simulink model "Simulink_Validation_Two_Bus_OPF_DER_Constraints"  (R2023b)
settings: Solver=ode4  StartTime=0.0  StopTime=1  FixedStep=1e-6  RelTol=1e-3  EnableMultiTasking=on
libraries: spsRMSLib x7, rtlab x3, spsControlledCurrentSourceLib x3, spsThreePhaseParallelRLCLoadLib x3, spsLoadFlowBusLib x2, spsThreePhaseVIMeasurementLib x2, SignalEditorBlockLib x2, eeGeneralControl x1, spsGroundLib x1, spsThreePhasePISectionLineLib x1, spsThreePhaseSourceLib x1, spsThreePhaseDynamicLoadLib x1
Description:
  | Model of a simple control system for use iin training.
settings Model: Creator=Paul Baracos  LastModifiedBy=Ali
settings SolverCC: AlgebraicLoopSolver=TrustRegion  AutoInsertRateTranBlk=on
settings DataIOCC: LimitDataPoints=on  SaveFormat=Array  SignalLoggingSaveFormat=ModelDataLogs  SaveOutput=off  SaveTime=off  ReturnWorkspaceOutputs=off  SignalLoggingName=sigsOut
settings OptimizationCC: BlockReduction=off  BooleanDataType=off  OptimizeBlockIOStorage=off  BufferReuse=off  ExpressionFolding=off  LocalBlockOutputs=off  InitFltsAndDblsToZero=on  LifeSpan=inf
settings DebuggingCC: SaveWithParameterizedLinksMsg=none  UnderspecifiedInitializationDetection=Classic  MergeDetectMultiDrivingBlocksExec=none  SignalResolutionControl=TryResolveAllWithWarning  MultiTaskDSMMsg=warning  MultiTaskCondExecSysMsg=none  FcnCallInpInsideContextMsg=warning  SFUnexpectedBacktrackingDiag=warning  SFNoUnconditionalDefaultTransitionDiag=warning  SFExecutionAtInitializationDiag=none  ArithmeticOperatorsInVariantConditions=warning
settings HardwareCC: ProdBitPerPointer=32  ProdBitPerSizeT=32  ProdBitPerPtrDiffT=32  ProdLargestAtomicFloat=None  ProdIntDivRoundTo=Undefined  ProdEndianess=Unspecified  ProdWordSize=32  ProdHWDeviceType=32-bit Generic  TargetUnknown=on
settings ModelReferenceCC: EnableRefExpFcnMdlSchedulingChecks=on  PropagateSignalLabelsOutOfModel=off
settings SFSimCC: SimUseLocalCustomCode=off  CustomCodeUndefinedFunction=UseInterfaceOnly
settings RTWCC: RTWUseLocalCustomCode=off  DLArmComputeVersion=19.05
settings CodeAppCC: StateflowObjectComments=on
settings GRTTargetCC: TargetFcnLib=ansi_tfl_tmw.mat  TargetLangStandard=C89/C90 (ANSI)  CombineOutputUpdateFcns=off  GRTInterface=on
settings ConfigComp: CovMetricSettings=dw  CovSaveCumulativeToWorkspaceVar=on  CovSaveSingleToWorkspaceVar=on  CovExternalEMLEnable=off

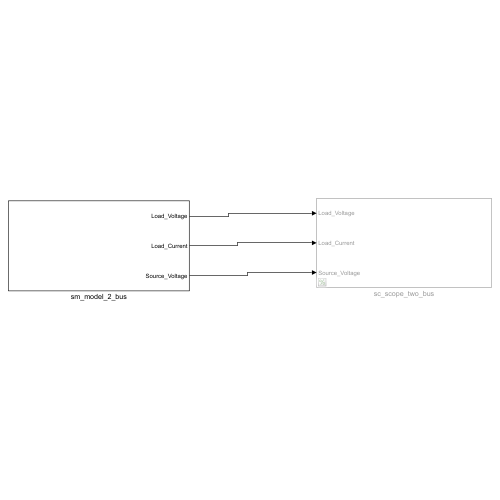
[thumbnail: Simulink's stored preview of the top-level diagram]
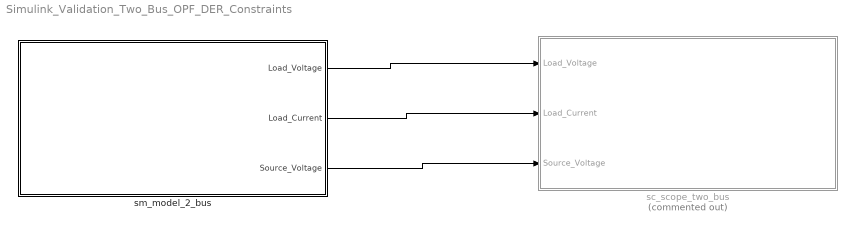
== system Simulink_Validation_Two_Bus_OPF_DER_Constraints ==
  sc_scope_two_bus : Subsystem  Commented=on
  sm_model_2_bus : Subsystem
  wires:
  sm_model_2_bus/1(Load_Voltage) -> sc_scope_two_bus/1(Load_Voltage)
  sm_model_2_bus/2(Load_Current) -> sc_scope_two_bus/2(Load_Current)
  sm_model_2_bus/3(Source_Voltage) -> sc_scope_two_bus/3(Source_Voltage)

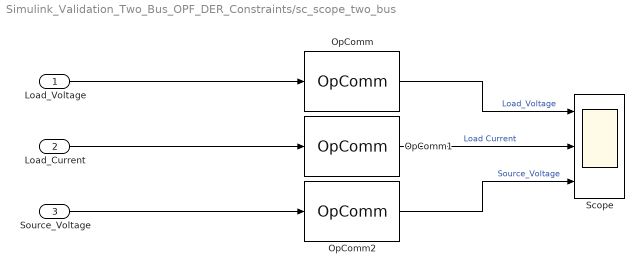
== system Simulink_Validation_Two_Bus_OPF_DER_Constraints/sc_scope_two_bus ==
  Load_Voltage : Inport
  Load_Current : Inport  Port=2
  Source_Voltage : Inport  Port=3
  OpComm : rtlab/OpComm  nbport=1  groupe_acq=1  subsys_rate=0  st=0  Synchronization=on  Interpolation=on  Threshold=1.0  Missed_Data=off  Sim_Time=off  Samples=off  dynSigOut=off  from_console=0  warning_done=off  writeOpCommFile=off  Offset=off
  OpComm1 : rtlab/OpComm  nbport=1  groupe_acq=2  subsys_rate=0  st=0  Synchronization=on  Interpolation=on  Threshold=1.0  Missed_Data=off  Sim_Time=off  Samples=off  dynSigOut=off  from_console=0  warning_done=off  writeOpCommFile=off  Offset=off
  OpComm2 : rtlab/OpComm  nbport=1  groupe_acq=3  subsys_rate=0  st=0  Synchronization=on  Interpolation=on  Threshold=1.0  Missed_Data=off  Sim_Time=off  Samples=off  dynSigOut=off  from_console=0  warning_done=off  writeOpCommFile=off  Offset=off
  Scope : Scope  NumInputPorts=3
  wires:
  OpComm/1 -> Scope/1  "Load_Voltage"
  Load_Voltage/1 -> OpComm/1
  OpComm2/1 -> Scope/3  "Source_Voltage"
  Source_Voltage/1 -> OpComm2/1
  OpComm1/1 -> Scope/2  "Load Current"
  Load_Current/1 -> OpComm1/1

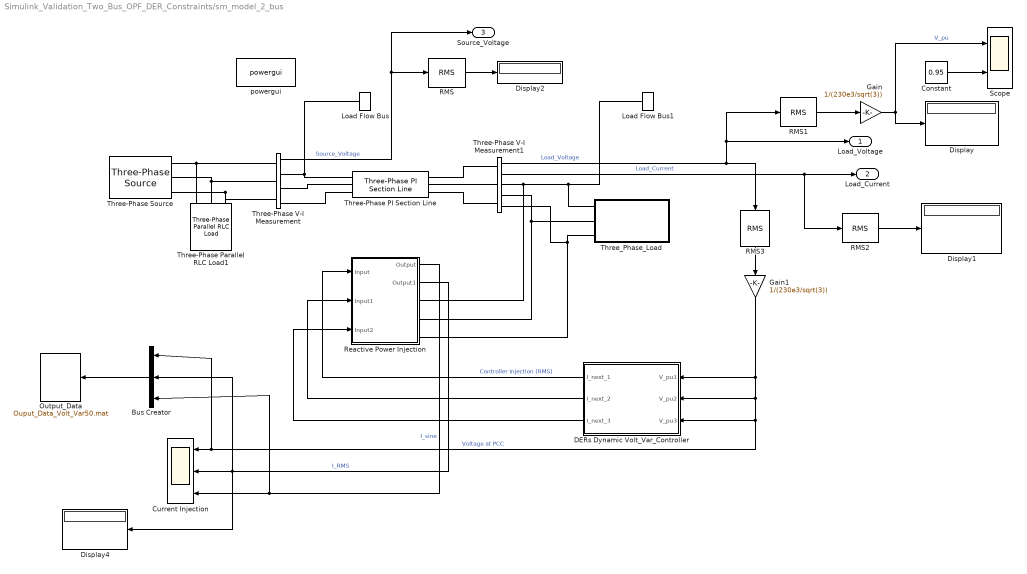
== system Simulink_Validation_Two_Bus_OPF_DER_Constraints/sm_model_2_bus ==
  Bus Creator : BusCreator  Inputs=3
  Constant : Constant  Value=0.95
  Current Injection : Scope  NumInputPorts=3
  DERs Dynamic Volt_Var_Controller : Subsystem
  Display{,1..2,4} (4 alike) : Display
  Gain : Gain  Gain=1/(230e3/sqrt(3))
  Gain1 : Gain  Gain=1/(230e3/sqrt(3))
  Load Flow Bus : spsLoadFlowBusLib/Load Flow Bus  LConnTagsString=a  Phases=single  Connectors=on one side  ID=BUS_1  Vbase=230e3  Vref=1.05  Vangle=0  VLF=1.05  VLFb=1  VLFc=1  angleLF=0  angleLFb=0  angleLFc=0
  Load Flow Bus1 : spsLoadFlowBusLib/Load Flow Bus  LConnTagsString=a  Phases=single  Connectors=on one side  ID=BUS_2  Vbase=230e3  Vref=0.957  Vangle=-11.19  VLF=0.9586  VLFb=1  VLFc=1  angleLF=-11.15  angleLFb=0  angleLFc=0
  Output_Data : ToFile  Filename=Ouput_Data_Volt_Var50.mat  MatrixName=results  SaveFormat=Timeseries
  RMS : spsRMSLib/RMS  TrueRMS=on  Freq=60  RMSInit=120  Ts=0
  RMS1 : spsRMSLib/RMS  TrueRMS=on  Freq=60  RMSInit=120  Ts=0
  RMS2 : spsRMSLib/RMS  TrueRMS=on  Freq=60  RMSInit=120  Ts=0
  RMS3 : spsRMSLib/RMS  TrueRMS=on  Freq=60  RMSInit=230e3/sqrt(3)  Ts=1e-4
  Reactive Power Injection : Subsystem
  Scope : Scope  NumInputPorts=2
  Three-Phase PI Section Line : spsThreePhasePISectionLineLib/Three-Phase PI Section Line  LConnTagsString=a|b|c  RConnTagsString=A|B|C  Length=10  Frequency=60  Resistances=[ 0.528 5.29]  Inductances="[ 0.0140  0.1404]"  Capacitances=[12.84e-9 7.751e-9]
  Three-Phase Parallel RLC Load1 : spsThreePhaseParallelRLCLoadLib/Three-Phase Parallel RLC Load  LConnTagsString=A|B|C  Configuration=Y (grounded)  NominalVoltage=(230000)*1.05  Vabc=[1e3 1e3 1e3]  Vabcp=[1e3 1e3 1e3]  NominalFrequency=60  UnbalancedPower=off  ActivePower=100000000  InductivePower=0  CapacitivePower=0  Pabc=[10e3 9e3 11e3]  QLabc=[100 90 110]  QCabc=[100 90 110]  Pabcp=[10e3 9e3 11e3]  QLabcp=[100 90 110]  QCabcp=[100 90 110]  Measurements=None  LoadType=constant PQ
  Three-Phase V-I Measurement : spsThreePhaseVIMeasurementLib/Three-Phase V-I Measurement  VoltageMeasurement=phase-to-phase  SetLabelV=off  LabelV=Vabc  Vpu=off  VpuLL=off  CurrentMeasurement=no  SetLabelI=off  LabelI=Iabc  Ipu=off  Pbase=100e6  Vbase=500e3  OutputType=Complex  PhasorSimulation=off  PSBequivalent=0
  Three-Phase V-I Measurement1 : spsThreePhaseVIMeasurementLib/Three-Phase V-I Measurement  VoltageMeasurement=phase-to-ground  SetLabelV=off  LabelV=Vabc  Vpu=off  VpuLL=off  CurrentMeasurement=yes  SetLabelI=off  LabelI=Iabc  Ipu=off  Pbase=100e6  Vbase=500e3  OutputType=Complex  PhasorSimulation=off  PSBequivalent=0
  Three-Phase Source : spsThreePhaseSourceLib/Three-Phase Source  InternalConnection=Yg  VoltagePhases=off  Voltage=(230000)*1.06591  PhaseAngle=1.762  Voltage_phases=[25e3 25e3 25e3]/sqrt(3)  PhaseAngles_phases=[0 -120 +120]  Frequency=60  NonIdealSource=on  SpecifyImpedance=off  Resistance=0.8929  Inductance=16.58e-3  ShortCircuitLevel=100e6  BaseVoltage=230e3  XRratio=7  BusType=swing  Pref=304.6  Qref=0  Prefabc=[10e3, 10e3, 10e3]  Qrefabc=[0, 0, 0]  Qmin=-200  Qmax=200
  Three_Phase_Load : Subsystem
  powergui : spspowerguiLib/powergui  Priority=1  SimulationMode=Discrete  SampleTime=1e-6  frequency=60  Iterations=50  frequencyindice=0  Pbase=100e6  ErrMax=1e-4  UnitsV=kV  UnitsW=MW  buscounter=0  FunctionMessages=off  echomessages=off  EnableUseOfTLC=off  CurrentSourceSwitches=off  DisableSnubberDevices=off  DisableRonSwitches=off  DisableVfSwitches=off  DisplayEquations=off  AutomaticDiscreteSolvers=off  SolverType=Tustin/Backward Euler (TBE)  Interpol=off  ExternalGateDelay=off  methode=off  Ts=100  x0status=blocks  SPID=on  SwTol=0  HookPort=off  NonlinearTolerance=1e-4  nMaxIteration=100  ContinueOnMaxIteration=off  RestoreLinks=warning  ResistiveCurrentMeasurement=off  Frange=[0:2:500]  Ylog=off  Xlog=on  ShowGrid=off  save=off  variable=ZData  structure=0  ZoomFFT=off  StartTime=0.0  cycles=1  DisplayStyle=1  fundamental=60  FreqAxis=off  MaxFrequency=1000  frequencyindicesteady=1  RmsSteady=1  display=off
  Load_Voltage : Outport
  Load_Current : Outport  Port=2
  Source_Voltage : Outport  Port=3
  wires:
  RMS1/1 -> Gain/1
  Three-Phase V-I Measurement1/1 -> RMS3/1, RMS1/1, Load_Voltage/1  "Load_Voltage"
  RMS2/1 -> Display1/1
  RMS/1 -> Display2/1
  Three-Phase V-I Measurement/1 -> Source_Voltage/1, RMS/1  "Source_Voltage"
  Three-Phase V-I Measurement1/2 -> RMS2/1, Load_Current/1  "Load_Current"
  Constant/1 -> Scope/2
  Gain/1 -> Display/1, Scope/1  "V_pu"
  RMS3/1 -> Gain1/1
  Reactive Power Injection/1(Output) -> Bus Creator/3, Current Injection/3  "I_sine"
  Gain1/1 -> Bus Creator/1, Current Injection/1, DERs Dynamic Volt_Var_Controller/3(V_pu3), DERs Dynamic Volt_Var_Controller/2(V_pu2), DERs Dynamic Volt_Var_Controller/1(V_pu1)  "Voltage at PCC"
  DERs Dynamic Volt_Var_Controller/1(I_next_1) -> Reactive Power Injection/1(Input)  "Controller Injection (RMS)"
  DERs Dynamic Volt_Var_Controller/2(I_next_2) -> Reactive Power Injection/2(Input1)
  DERs Dynamic Volt_Var_Controller/3(I_next_3) -> Reactive Power Injection/3(Input2)
  Reactive Power Injection/2(Output1) -> Bus Creator/2, Display4/1, Current Injection/2  "I_RMS"
  Bus Creator/1 -> Output_Data/1
  connections:
  Load Flow Bus1/LConn1 -- Three_Phase_Load/LConn1 -- Reactive Power Injection/RConn1 -- Three-Phase V-I Measurement1/RConn1
  Three-Phase V-I Measurement/RConn3 -- Three-Phase PI Section Line/LConn3
  Three-Phase Parallel RLC Load1/LConn1 -- Three-Phase V-I Measurement/LConn1 -- Three-Phase Source/RConn1
  Three-Phase V-I Measurement/RConn1 -- Load Flow Bus/LConn1 -- Three-Phase PI Section Line/LConn1
  Three-Phase Parallel RLC Load1/LConn3 -- Three-Phase V-I Measurement/LConn3 -- Three-Phase Source/RConn3
  Three-Phase Parallel RLC Load1/LConn2 -- Three-Phase Source/RConn2 -- Three-Phase V-I Measurement/LConn2
  Three-Phase V-I Measurement/RConn2 -- Three-Phase PI Section Line/LConn2
  Three-Phase V-I Measurement1/LConn2 -- Three-Phase PI Section Line/RConn2
  Three-Phase V-I Measurement1/LConn3 -- Three-Phase PI Section Line/RConn3
  Three-Phase V-I Measurement1/LConn1 -- Three-Phase PI Section Line/RConn1
  Three-Phase V-I Measurement1/RConn2 -- Reactive Power Injection/RConn2 -- Three_Phase_Load/LConn2
  Three-Phase V-I Measurement1/RConn3 -- Reactive Power Injection/RConn3 -- Three_Phase_Load/LConn3

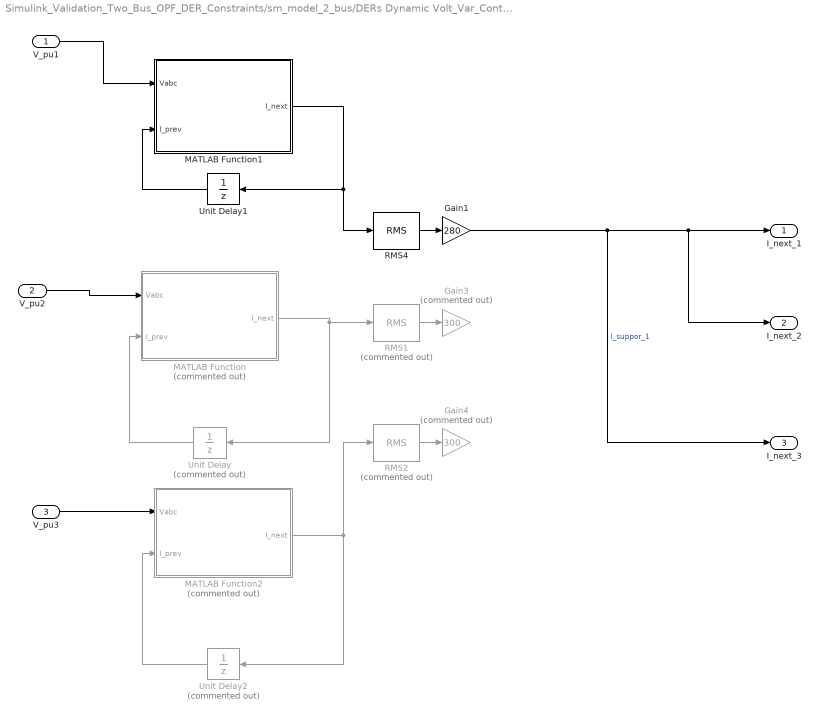
== system Simulink_Validation_Two_Bus_OPF_DER_Constraints/sm_model_2_bus/DERs Dynamic Volt_Var_Controller ==
  V_pu1 : Inport
  V_pu2 : Inport  Port=2
  V_pu3 : Inport  Port=3
  Gain1 : Gain  Gain=280
  Gain3 : Gain  Commented=on  Gain=300
  Gain4 : Gain  Commented=on  Gain=300
  MATLAB Function : MATLAB Function  Commented=on  TreatAsAtomicUnit=on
  MATLAB Function1 : MATLAB Function  TreatAsAtomicUnit=on
  MATLAB Function2 : MATLAB Function  Commented=on  TreatAsAtomicUnit=on
  RMS1 : spsRMSLib/RMS  Commented=on  TrueRMS=on  Freq=60  RMSInit=0.1  Ts=1e-4
  RMS2 : spsRMSLib/RMS  Commented=on  TrueRMS=on  Freq=60  RMSInit=0.1  Ts=1e-4
  RMS4 : spsRMSLib/RMS  TrueRMS=on  Freq=60  RMSInit=0  Ts=1e-4
  Unit Delay : UnitDelay  Commented=on  InitialCondition=0.01  SampleTime=1e-4  HasFrameUpgradeWarning=on
  Unit Delay1 : UnitDelay  SampleTime=1e-4  HasFrameUpgradeWarning=on
  Unit Delay2 : UnitDelay  Commented=on  InitialCondition=0.01  SampleTime=1e-4  HasFrameUpgradeWarning=on
  I_next_1 : Outport
  I_next_2 : Outport  Port=2
  I_next_3 : Outport  Port=3
  wires:
  Unit Delay/1 -> MATLAB Function/2(I_prev)
  V_pu2/1 -> MATLAB Function/1(Vabc)
  MATLAB Function/1(I_next) -> Unit Delay/1, RMS1/1
  MATLAB Function1/1(I_next) -> RMS4/1, Unit Delay1/1
  V_pu1/1 -> MATLAB Function1/1(Vabc)
  Unit Delay1/1 -> MATLAB Function1/2(I_prev)
  MATLAB Function2/1(I_next) -> Unit Delay2/1, RMS2/1
  V_pu3/1 -> MATLAB Function2/1(Vabc)
  Unit Delay2/1 -> MATLAB Function2/2(I_prev)
  RMS4/1 -> Gain1/1
  RMS1/1 -> Gain3/1
  RMS2/1 -> Gain4/1
  Gain1/1 -> I_next_3/1, I_next_2/1, I_next_1/1  "I_suppor_1"

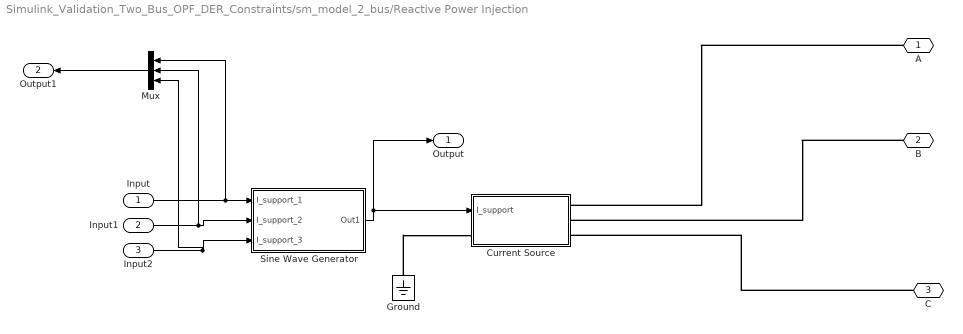
== system Simulink_Validation_Two_Bus_OPF_DER_Constraints/sm_model_2_bus/Reactive Power Injection ==
  Input : Inport
  Input1 : Inport  Port=2
  Input2 : Inport  Port=3
  Current Source : Subsystem
  Ground : spsGroundLib/Ground  LConnTagsString=a
  Mux : Mux  Inputs=3
  Sine Wave Generator : Subsystem
  A : PMIOPort  Side=Right
  B : PMIOPort  Port=2  Side=Right
  C : PMIOPort  Port=3  Side=Right
  Output : Outport
  Output1 : Outport  Port=2
  wires:
  Sine Wave Generator/1(Out1) -> Output/1, Current Source/1(I_support)
  Input/1 -> Mux/1, Sine Wave Generator/1(I_support_1)
  Input1/1 -> Mux/2, Sine Wave Generator/2(I_support_2)
  Input2/1 -> Mux/3, Sine Wave Generator/3(I_support_3)
  Mux/1 -> Output1/1
  connections:
  Ground/LConn1 -- Current Source/LConn1
  A/RConn1 -- Current Source/RConn1
  B/RConn1 -- Current Source/RConn2
  C/RConn1 -- Current Source/RConn3

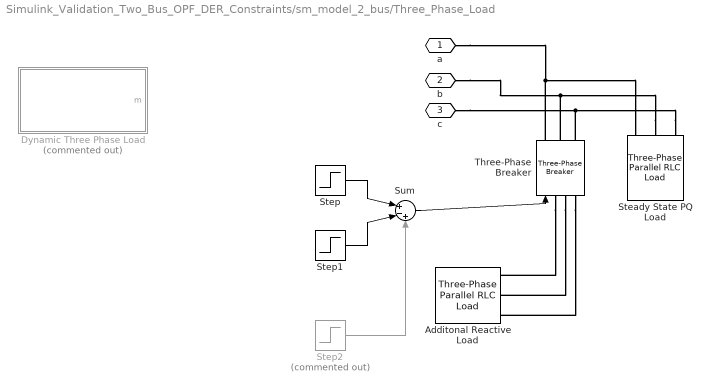
== system Simulink_Validation_Two_Bus_OPF_DER_Constraints/sm_model_2_bus/Three_Phase_Load ==
  Additonal Reactive Load : spsThreePhaseParallelRLCLoadLib/Three-Phase Parallel RLC Load  LConnTagsString=A|B|C  Configuration=Y (grounded)  NominalVoltage=(230000)*0.95859  Vabc=[230e3/sqrt(3) 230e3/sqrt(3) 230e3/sqrt(3)]  Vabcp=[1e3 1e3 1e3]  NominalFrequency=60  UnbalancedPower=off  ActivePower=0  InductivePower=25000000  CapacitivePower=0  Pabc=[0 0 0]  QLabc=[10e6 10e6 10e6]  QCabc=[0 0 0]  Pabcp=[10e3 9e3 11e3]  QLabcp=[100 90 110]  QCabcp=[100 90 110]  Measurements=None  LoadType=constant PQ
  Dynamic Three Phase Load : Subsystem  Commented=on
  Steady State PQ Load : spsThreePhaseParallelRLCLoadLib/Three-Phase Parallel RLC Load  LConnTagsString=A|B|C  Configuration=Y (grounded)  NominalVoltage=(230000)*0.95859  Vabc=[230e3/sqrt(3)*0.95859 230e3/sqrt(3)*0.95859 230e3/sqrt(3)*0.95859]  Vabcp=[1e3 1e3 1e3]  NominalFrequency=60  UnbalancedPower=off  ActivePower=200000000  InductivePower=50000000  CapacitivePower=0  Pabc=[10e3 10e3 10e3]  QLabc=[40 40 30]  QCabc=[0 0 0]  Pabcp=[10e3 9e3 11e3]  QLabcp=[100 90 110]  QCabcp=[100 90 110]  Measurements=None  LoadType=constant PQ
  Step : Step  Time=0.3  SampleTime=0
  Step1 : Step  Time=0.7  SampleTime=0
  Step2 : Step  Commented=on  Time=0.8  SampleTime=0
  Sum : Sum  Inputs=|+-+
  Three-Phase Breaker : spsThreePhaseBreakerLib/Three-Phase Breaker  InitialState=open  SwitchA=on  SwitchB=on  SwitchC=on  SwitchTimes="[1/60  5/60]"  External=on  BreakerResistance=0.01  SnubberResistance=1e6  SnubberCapacitance=inf  Measurements=None
  a : PMIOPort  Side=Left
  b : PMIOPort  Port=2  Side=Left
  c : PMIOPort  Port=3  Side=Left
  wires:
  Step1/1 -> Sum/2
  Step/1 -> Sum/1
  Sum/1 -> Three-Phase Breaker/1
  Step2/1 -> Sum/3
  connections:
  Steady State PQ Load/LConn3 -- c/RConn1 -- Three-Phase Breaker/RConn3
  Three-Phase Breaker/LConn3 -- Additonal Reactive Load/LConn3
  Steady State PQ Load/LConn2 -- b/RConn1 -- Three-Phase Breaker/RConn2
  Three-Phase Breaker/LConn2 -- Additonal Reactive Load/LConn2
  Three-Phase Breaker/LConn1 -- Additonal Reactive Load/LConn1
  Three-Phase Breaker/RConn1 -- a/RConn1 -- Steady State PQ Load/LConn1

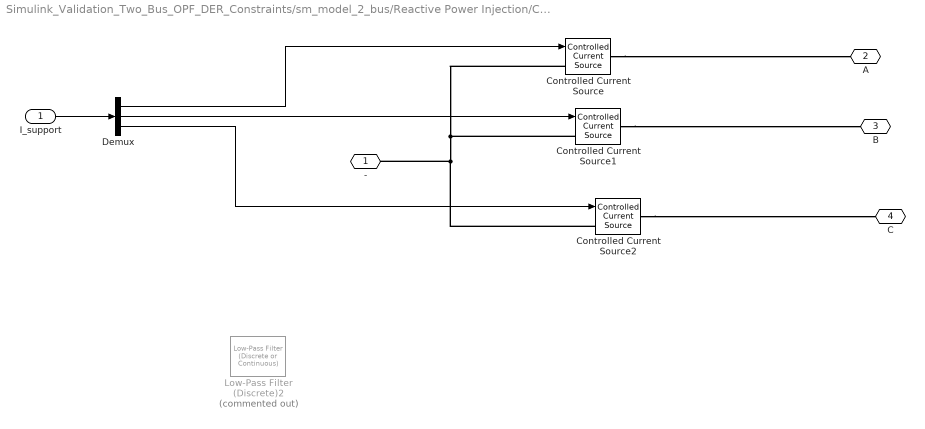
== system Simulink_Validation_Two_Bus_OPF_DER_Constraints/sm_model_2_bus/Reactive Power Injection/Current Source ==
  I_support : Inport
  Controlled Current Source : spsControlledCurrentSourceLib/Controlled Current Source  Initialize=off  Source_Type=AC  Amplitude=28  Phase=0  Frequency=60  Measurements=Current
  Controlled Current Source1 : spsControlledCurrentSourceLib/Controlled Current Source  Initialize=off  Source_Type=AC  Amplitude=28  Phase=-120  Frequency=60  Measurements=None
  Controlled Current Source2 : spsControlledCurrentSourceLib/Controlled Current Source  Initialize=off  Source_Type=AC  Amplitude=28  Phase=120  Frequency=60  Measurements=None
  Demux : Demux  Outputs=3
  Low-Pass Filter (Discrete)2 : eeGeneralControl/Low-Pass Filter (Discrete or Continuous)  Commented=on  K=1  T=0.5  B=inf  A=-inf  init_option=Specify as parameter  x0=0  Ts=1e-6
  - : PMIOPort  Side=Left
  A : PMIOPort  Port=2  Side=Right
  B : PMIOPort  Port=3  Side=Right
  C : PMIOPort  Port=4  Side=Right
  wires:
  I_support/1 -> Demux/1
  Demux/2 -> Controlled Current Source1/1
  Demux/1 -> Controlled Current Source/1
  Demux/3 -> Controlled Current Source2/1
  connections:
  Controlled Current Source/LConn1 -- Controlled Current Source1/LConn1 -- Controlled Current Source2/LConn1 -- -/RConn1
  Controlled Current Source1/RConn1 -- B/RConn1
  Controlled Current Source2/RConn1 -- C/RConn1
  Controlled Current Source/RConn1 -- A/RConn1

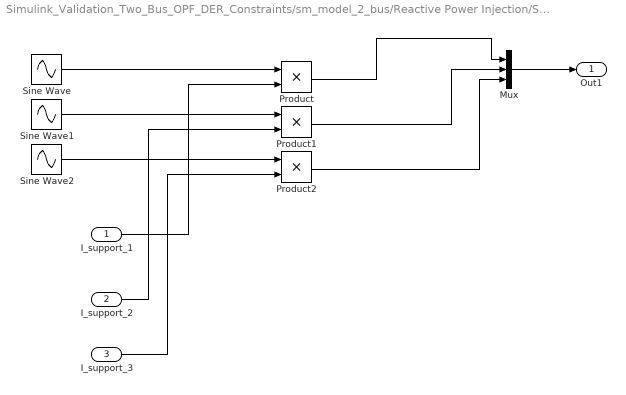
== system Simulink_Validation_Two_Bus_OPF_DER_Constraints/sm_model_2_bus/Reactive Power Injection/Sine Wave Generator ==
  I_support_1 : Inport
  I_support_2 : Inport  Port=2
  I_support_3 : Inport  Port=3
  Mux : Mux  Inputs=3
  Product : Product
  Product1 : Product
  Product2 : Product
  Sine Wave : Sin  Frequency=2*pi*60  SampleTime=1e-6
  Sine Wave1 : Sin  Frequency=2*pi*60  Phase=-(2/3) *pi  SampleTime=1e-6
  Sine Wave2 : Sin  Frequency=2*pi*60  Phase=(2/3) * pi  SampleTime=1e-6
  Out1 : Outport
  wires:
  Mux/1 -> Out1/1
  Sine Wave/1 -> Product/1
  Sine Wave2/1 -> Product2/1
  Product1/1 -> Mux/2
  Product2/1 -> Mux/3
  Product/1 -> Mux/1
  Sine Wave1/1 -> Product1/1
  I_support_1/1 -> Product/2
  I_support_2/1 -> Product1/2
  I_support_3/1 -> Product2/2

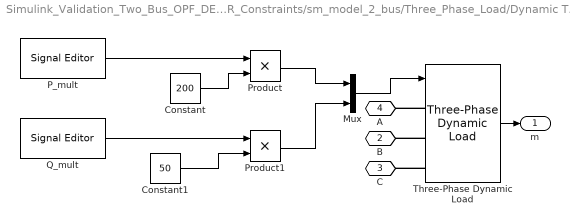
== system Simulink_Validation_Two_Bus_OPF_DER_Constraints/sm_model_2_bus/Three_Phase_Load/Dynamic Three Phase Load ==
  Constant : Constant  Value=200
  Constant1 : Constant  Value=50
  Mux : Mux  Inputs=2
  P_mult : SignalEditorBlockLib/Signal Editor  FileName=P_mult.mat  ActiveScenario=P_mult  ActiveSignal=Signal  IsBus=off  OutputBusObjectStr=Bus: BusObject  SampleTime=0  Interpolate=off  ZeroCross=off  OutputAfterFinalValue=Setting to zero  Unit=inherit  PreserveSignalName=on  ApplySigPropsToAllScenarios=on  ApplySigPropsToAllSignals=off
  Product : Product
  Product1 : Product
  Q_mult : SignalEditorBlockLib/Signal Editor  FileName=Q_mult.mat  ActiveScenario=Q_mult  ActiveSignal=Signal 1  IsBus=off  OutputBusObjectStr=Bus: BusObject  SampleTime=0  Interpolate=off  ZeroCross=off  OutputAfterFinalValue=Setting to zero  Unit=inherit  PreserveSignalName=on  ApplySigPropsToAllScenarios=on  ApplySigPropsToAllSignals=off
  Three-Phase Dynamic Load : spsThreePhaseDynamicLoadLib/Three-Phase Dynamic Load  NominalVoltage=[ 230e3 60 ]  ActiveReactivePowers=[200e6 50e6]  PositiveSequence=[0.958 11.8]  ExternalControl=on  NpNq=[1.3 2]  TimeConstants="[0  0  0  0]"  MinimumVoltage=0.7  Tfilter=1e-4  LoadFlowParameters=[4,0,0,0,0]
      settings: LibrarySourceBlock=|
      | sps_lib/Passives/Three-Phase
      | Dynamic Load
  B : PMIOPort  Port=2  Side=Left
  C : PMIOPort  Port=3  Side=Left
  A : PMIOPort  Port=4  Side=Left
  m : Outport
  wires:
  Constant/1 -> Product/2
  Product/1 -> Mux/1
  P_mult/1 -> Product/1
  Constant1/1 -> Product1/2
  Product1/1 -> Mux/2
  Mux/1 -> Three-Phase Dynamic Load/1
  Q_mult/1 -> Product1/1
  Three-Phase Dynamic Load/1 -> m/1
  connections:
  Three-Phase Dynamic Load/LConn3 -- C/RConn1
  Three-Phase Dynamic Load/LConn2 -- B/RConn1
  Three-Phase Dynamic Load/LConn1 -- A/RConn1

== matlab function Simulink_Validation_Two_Bus_OPF_DER_Constraints/sm_model_2_bus/DERs Dynamic Volt_Var_Controller/MATLAB Function ==
  data: Vabc input; I_prev input; I_next output
function I_next = DERs_Dynamics(Vabc, I_prev)
% DERs_Dynamics: one‐step update for DER reactive current injection
% using pre-identified coefficients in voltage intervals

  persistent intervals coeffs Ts
  if isempty(intervals)
    Ts = 1e-4;  % time step

    % Voltage intervals
    intervals = [
      0.89, 0.90;
      0.90, 0.91;
      0.91, 0.92;
      0.92, 0.93;
      0.93, 0.94;
      0.94, 0.95;
      0.95, 0.96;
      0.96, 0.97;
      0.97, 0.98;
      0.98, 0.99;
      0.99, 1.00;
      1.00, 1.01;
      1.01, 1.02;
      1.02, 1.03;
      1.03, 1.04;
      1.04, 1.05;
      1.05, 1.06;
      1.06, 1.07;
      1.07, 1.08;
      1.08, 1.09
    ];

    % Coefficients [C, A, B] (as provided by you)
    coeffs = [... % same as what you pasted above
       0.001343,  0.124496,  0.000255;
      -0.021229,  0.760987,  0.000004;
      -0.046148,  1.014878,  0.000006;
      -0.091656,  1.336320,  0.000001;
      -0.130297,  1.533759,  0.000001;
      -0.075666,  1.327522,  0.000003;
       0.327990, -0.041007, -0.000031;
       0.321990, -0.033553, -0.000072;
       0.392218, -0.206472, -0.000020;
       0.042008,  0.564053,  0.000014;
      -0.531410,  1.719224, -0.000001;
      -0.727948,  2.080821, -0.000001;
      -0.713179,  2.055411,  0.000001;
      -0.822510,  2.223830, -0.000001;
      -0.764602,  2.142240,  0.000001;
      -0.584279,  1.902945,  0.000001;
       0.086320,  1.069394, -0.000005;
       0.955678,  0.048408, -0.000306;
       1.205022, -0.231621,  0.000012;
       1.129212, -0.148427, -0.000024
    ];
  end

  % Assume balanced Vabc, take magnitude of phase A
  V = abs(Vabc(2));

  % Find interval
  idx = find(V >= intervals(:,1) & V < intervals(:,2), 1);
  if isempty(idx)
    if V < intervals(1,1)
      idx = 1;
    else
      idx = size(intervals,1);
    end
  end

  % Extract coefficients
  C = coeffs(idx,1);
  A = coeffs(idx,2);
  B = coeffs(idx,3);

  % Prevent division by zero or overflow
  if abs(B) < 1e-6
    I_next = I_prev;  % hold previous value if dynamics are numerically unstable
    return;
  end

  % Compute discrete-time update (Backward Euler)
  D = Ts / B;
  den = (1 - D);

  if abs(den) < 1e-6
    I_next = I_prev;  % avoid division by near-zero
    return;
  end

  alpha = 1 / den;
  beta  = -D * A / den;
  gamma = -D * C / den;

 % I_next = I_prev + beta * V + gamma;
   I_next = alpha * I_prev + beta * V + gamma;
end

== matlab function Simulink_Validation_Two_Bus_OPF_DER_Constraints/sm_model_2_bus/DERs Dynamic Volt_Var_Controller/MATLAB Function2 ==
  data: Vabc input; I_prev input; I_next output
function I_next = DERs_Dynamics(Vabc, I_prev)
% DERs_Dynamics: one‐step update for DER reactive current injection
% using pre-identified coefficients in voltage intervals

  persistent intervals coeffs Ts
  if isempty(intervals)
    Ts = 1e-4;  % time step

    % Voltage intervals
    intervals = [
      0.89, 0.90;
      0.90, 0.91;
      0.91, 0.92;
      0.92, 0.93;
      0.93, 0.94;
      0.94, 0.95;
      0.95, 0.96;
      0.96, 0.97;
      0.97, 0.98;
      0.98, 0.99;
      0.99, 1.00;
      1.00, 1.01;
      1.01, 1.02;
      1.02, 1.03;
      1.03, 1.04;
      1.04, 1.05;
      1.05, 1.06;
      1.06, 1.07;
      1.07, 1.08;
      1.08, 1.09
    ];

    % Coefficients [C, A, B] (as provided by you)
    coeffs = [... % same as what you pasted above
       0.001343,  0.124496,  0.000255;
      -0.021229,  0.760987,  0.000004;
      -0.046148,  1.014878,  0.000006;
      -0.091656,  1.336320,  0.000001;
      -0.130297,  1.533759,  0.000001;
      -0.075666,  1.327522,  0.000003;
       0.327990, -0.041007, -0.000031;
       0.321990, -0.033553, -0.000072;
       0.392218, -0.206472, -0.000020;
       0.042008,  0.564053,  0.000014;
      -0.531410,  1.719224, -0.000001;
      -0.727948,  2.080821, -0.000001;
      -0.713179,  2.055411,  0.000001;
      -0.822510,  2.223830, -0.000001;
      -0.764602,  2.142240,  0.000001;
      -0.584279,  1.902945,  0.000001;
       0.086320,  1.069394, -0.000005;
       0.955678,  0.048408, -0.000306;
       1.205022, -0.231621,  0.000012;
       1.129212, -0.148427, -0.000024
    ];
  end

  % Assume balanced Vabc, take magnitude of phase A
  V = abs(Vabc(3));

  % Find interval
  idx = find(V >= intervals(:,1) & V < intervals(:,2), 1);
  if isempty(idx)
    if V < intervals(1,1)
      idx = 1;
    else
      idx = size(intervals,1);
    end
  end

  % Extract coefficients
  C = coeffs(idx,1);
  A = coeffs(idx,2);
  B = coeffs(idx,3);

  % Prevent division by zero or overflow
  if abs(B) < 1e-6
    I_next = I_prev;  % hold previous value if dynamics are numerically unstable
    return;
  end

  % Compute discrete-time update (Backward Euler)
  D = Ts / B;
  den = (1 - D);

  if abs(den) < 1e-6
    I_next = I_prev;  % avoid division by near-zero
    return;
  end

  alpha = 1 / den;
  beta  = -D * A / den;
  gamma = -D * C / den;

 % I_next = I_prev + beta * V + gamma;
   I_next = alpha * I_prev + beta * V + gamma;
end

== matlab function Simulink_Validation_Two_Bus_OPF_DER_Constraints/sm_model_2_bus/DERs Dynamic Volt_Var_Controller/MATLAB Function1 ==
  data: Vabc input; I_prev input; I_next output
function I_next = DERs_Dynamics(Vabc, I_prev)
% DERs_Dynamics: one‐step update for DER reactive current injection
% using pre-identified coefficients in voltage intervals

  persistent intervals coeffs Ts
  if isempty(intervals)
    Ts = 1e-4;  % time step

    % Voltage intervals
    intervals = [
      0.89, 0.90;
      0.90, 0.91;
      0.91, 0.92;
      0.92, 0.93;
      0.93, 0.94;
      0.94, 0.96;
     % 0.95, 0.96;
      0.96, 0.97;
      0.97, 0.98;
      0.98, 0.99;
      0.99, 1.00;
      1.00, 1.01;
      1.01, 1.02;
      1.02, 1.03;
      1.03, 1.04;
      1.04, 1.05;
      1.05, 1.06;
      1.06, 1.07;
      1.07, 1.08;
      1.08, 1.09
    ];

    % Coefficients [C, A, B] (as provided by you)
    coeffs = [... % same as what you pasted above
       0.001343,  0.124496,  0.000255;
      -0.021229,  0.760987,  0.000004;
      -0.046148,  1.014878,  0.000006;
      -0.091656,  1.336320,  0.000001;
      -0.130297,  1.533759,  0.000001;
      -0.075666,  1.327522,  0.000003;
      % 0.327990, -0.041007, -0.000031;
       0.321990, -0.033553, -0.000072;
       0.392218, -0.206472, -0.000020;
       0.042008,  0.564053,  0.000014;
      -0.531410,  1.719224, -0.000001;
      -0.727948,  2.080821, -0.000001;
      -0.713179,  2.055411,  0.000001;
      -0.822510,  2.223830, -0.000001;
      -0.764602,  2.142240,  0.000001;
      -0.584279,  1.902945,  0.000001;
       0.086320,  1.069394, -0.000005;
       0.955678,  0.048408, -0.000306;
       1.205022, -0.231621,  0.000012;
       1.129212, -0.148427, -0.000024
    ];
  end

  % Assume balanced Vabc, take magnitude of phase A
  V = abs(Vabc(3));

  % Find interval
  idx = find(V >= intervals(:,1) & V < intervals(:,2), 1);
  if isempty(idx)
    if V < intervals(1,1)
      idx = 1;
    else
      idx = size(intervals,1);
    end
  end

  % Extract coefficients
  C = coeffs(idx,1);
  A = coeffs(idx,2);
  B = coeffs(idx,3);

  % Prevent division by zero or overflow
  if abs(B) < 1e-6
    I_next = I_prev;  % hold previous value if dynamics are numerically unstable
    return;
  end

  % Compute discrete-time update (Backward Euler)
  D = Ts / B;
  den = (1 - D);

  if abs(den) < 1e-6
    I_next = I_prev;  % avoid division by near-zero
    return;
  end

  alpha = 1 / den;
  beta  = -D * A / den;
  gamma = -D * C / den;

 % I_next = I_prev + beta * V + gamma;
   I_next = alpha * I_prev + beta * V + gamma;
end
